simulink library "AFCToolbox"  (R2025b)
settings: Solver=VariableStepAuto  StartTime=0.0  StopTime=10.0  RelTol=1e-3
undefined symbols (not defined in the file or in its folder): AFC5Toolbox_SimuMoudle, ax, ay, az, C_d, C_dm, C_m, C_t, Control, d, declination_table, dp0, dp1, dp2, dp3, dt, euler_0, g0, I_xyz, inclination_table, J_m, lmd_high, lmd_low, lp_acc_knoise, lp_acc_max, lp_acc_min, lp_acc_seed, lp_GPS_BL_max, lp_GPS_BL_min, lp_GPS_H_max, lp_GPS_H_min, lp_GPS_knoise, lp_GPS_seed, lp_GPS_vel_max, lp_GPS_vel_min, lp_gyro_knoise, lp_gyro_max, lp_gyro_min, lp_gyro_seed, lp_hf_vwind, lp_hs_vwind_interp, lp_kaerorho, lp_kaeroT, lp_kIxyz, lp_kmass, lp_momentx_A0, lp_momentx_Af, lp_momentx_ts, lp_momenty_A0, lp_momenty_Af, lp_momenty_ts, lp_momentz_A0, lp_momentz_Af, lp_momentz_ts, lp_vf_vwind, lp_vs_vwind_interp, lp_vwind_thetax, lp_vwind_thetaz, mass, MB_states ... (+52)
libraries: $bdroot x104, simulink x75, etargetslib x32, sharedtransform x13, simulink_extras x12, dspstat3 x11, aerolibconvert2 x9, aerolibtransform2 x3, aerolibutil x2, matrix_library x1
(part 8 of 11)

== system AFCToolbox/SimuMoudle/UAV/Forces & Moments/Parameters/Air Parameter1/Air Model/W zhishu ==
  note: 1
  note: 2
  note: 3
  note: 4
  note: 5
  note: 6
  note: 7
  note: 8
  Z : Inport
  1 : Switch  Threshold=11.0191  SaturateOnIntegerOverflow=off  InputSameDT=off
  2 : Switch  Threshold=20.0631  SaturateOnIntegerOverflow=off  InputSameDT=off
  3 : Switch  Threshold=32.1619  SaturateOnIntegerOverflow=off  InputSameDT=off
  4 : Switch  Threshold=47.3501  SaturateOnIntegerOverflow=off  InputSameDT=off
  5 : Switch  Threshold=51.4125  SaturateOnIntegerOverflow=off  InputSameDT=off
  6 : Switch  Threshold=71.8020  SaturateOnIntegerOverflow=off  InputSameDT=off
  7 : Switch  Threshold=86  SaturateOnIntegerOverflow=off  InputSameDT=off
  constant1 : Constant  Value=11.2011
  constant10 : Constant
  constant11 : Constant  Value=-13.2011
  constant4 : Constant  Value=16.0816
  constant6 : Constant
  constant7 : Constant  Value=4.2559
  constant8 : Constant
  constant9 : Constant  Value=-35.1629
  zhishu : Outport
  wires:
  constant7/1 -> 1/3
  constant8/1 -> 1/1
  constant9/1 -> 2/1
  1/1 -> 2/3
  constant11/1 -> 3/1
  2/1 -> 3/3
  constant10/1 -> 4/1
  3/1 -> 4/3
  constant1/1 -> 5/1
  4/1 -> 5/3
  constant4/1 -> 6/1
  5/1 -> 6/3
  constant6/1 -> 7/1
  6/1 -> 7/3
  Z/1 -> 2/2, 6/2, 7/2, 5/2, 1/2, 3/2, 4/2
  7/1 -> zhishu/1

== system AFCToolbox/SimuMoudle/UAV/Forces & Moments/Parameters/Air Parameter1/Air Model/W zhishu1 ==
  note: 8
  note: 7
  note: 6
  note: 5
  note: 4
  note: 3
  note: 2
  note: 1
  Z : Inport
  1 : Switch  Threshold=11.0191  SaturateOnIntegerOverflow=off  InputSameDT=off
  2 : Switch  Threshold=20.0631  SaturateOnIntegerOverflow=off  InputSameDT=off
  3 : Switch  Threshold=32.1619  SaturateOnIntegerOverflow=off  InputSameDT=off
  4 : Switch  Threshold=47.3501  SaturateOnIntegerOverflow=off  InputSameDT=off
  5 : Switch  Threshold=51.4125  SaturateOnIntegerOverflow=off  InputSameDT=off
  6 : Switch  Threshold=71.8020  SaturateOnIntegerOverflow=off  InputSameDT=off
  7 : Switch  Threshold=86  SaturateOnIntegerOverflow=off  InputSameDT=off
  constant1 : Constant  Value=12.2011
  constant10 : Constant
  constant11 : Constant  Value=-12.2011
  constant4 : Constant  Value=17.0816
  constant6 : Constant
  constant7 : Constant  Value=5.2559
  constant8 : Constant
  constant9 : Constant  Value=-34.1629
  zhishu : Outport
  wires:
  7/1 -> zhishu/1
  Z/1 -> 4/2, 3/2, 1/2, 5/2, 7/2, 6/2, 2/2
  6/1 -> 7/3
  constant6/1 -> 7/1
  5/1 -> 6/3
  constant4/1 -> 6/1
  4/1 -> 5/3
  constant1/1 -> 5/1
  3/1 -> 4/3
  constant10/1 -> 4/1
  2/1 -> 3/3
  constant11/1 -> 3/1
  1/1 -> 2/3
  constant9/1 -> 2/1
  constant8/1 -> 1/1
  constant7/1 -> 1/3

== system AFCToolbox/SimuMoudle/UAV/Forces & Moments/Parameters/Air Parameter1/Air Model/rho xishu ==
  note: 8
  note: 7
  note: 6
  note: 5
  note: 4
  note: 3
  note: 2
  note: 1
  note: 9
  Z : Inport
  1 : Switch  Threshold=11.0191  SaturateOnIntegerOverflow=off  InputSameDT=off
  2 : Switch  Threshold=20.0631  SaturateOnIntegerOverflow=off  InputSameDT=off
  3 : Switch  Threshold=32.1619  SaturateOnIntegerOverflow=off  InputSameDT=off
  4 : Switch  Threshold=47.3501  SaturateOnIntegerOverflow=off  InputSameDT=off
  5 : Switch  Threshold=51.4125  SaturateOnIntegerOverflow=off  InputSameDT=off
  6 : Switch  Threshold=71.8020  SaturateOnIntegerOverflow=off  InputSameDT=off
  7 : Switch  Threshold=86  SaturateOnIntegerOverflow=off  InputSameDT=off
  8 : Switch  Threshold=91  SaturateOnIntegerOverflow=off  InputSameDT=off
  constant1 : Constant  Value=2.5280e-4
  constant10 : Constant  Value=9.4920e-4
  constant11 : Constant  Value=3.2618e-3
  constant2 : Constant  Value=0
  constant4 : Constant  Value=1.7632e-5
  constant6 : Constant  Value=3.6411e-6
  constant7 : Constant
  constant8 : Constant  Value=1.5898e-1
  constant9 : Constant  Value=3.2722e-2
  xishu : Outport
  wires:
  Z/1 -> 4/2, 3/2, 1/2, 5/2, 6/2, 7/2, 8/2, 2/2
  6/1 -> 7/3
  constant6/1 -> 7/1
  5/1 -> 6/3
  constant4/1 -> 6/1
  4/1 -> 5/3
  constant1/1 -> 5/1
  3/1 -> 4/3
  constant10/1 -> 4/1
  2/1 -> 3/3
  constant11/1 -> 3/1
  1/1 -> 2/3
  constant9/1 -> 2/1
  constant8/1 -> 1/1
  constant7/1 -> 1/3
  constant2/1 -> 8/1
  7/1 -> 8/3
  8/1 -> xishu/1

== system AFCToolbox/基础导航算法模型库/ECL EKF/init_state/State_mag1/Subsystem1/Subsystem/round down1 ==
  lat : Inport
  Data Type Conversion2 : DataTypeConversion  OutDataTypeStr=single  SaturateOnIntegerOverflow=off  RndMeth=Floor
  Floor2 : Rounding
  rad_to_index2 : Gain  Gain=0.1  OutDataTypeStr=int32
  rad_to_index3 : Gain  Gain=10  OutDataTypeStr=int32
  min_lat : Outport
  wires:
  Floor2/1 -> rad_to_index3/1
  lat/1 -> rad_to_index2/1
  rad_to_index3/1 -> min_lat/1
  rad_to_index2/1 -> Data Type Conversion2/1
  Data Type Conversion2/1 -> Floor2/1

== system AFCToolbox/基础导航算法模型库/ECL EKF/init_state/State_mag1/Subsystem1/Subsystem/round down3 ==
  lon : Inport
  Data Type Conversion2 : DataTypeConversion  OutDataTypeStr=single  SaturateOnIntegerOverflow=off  RndMeth=Floor
  Floor2 : Rounding
  rad_to_index2 : Gain  Gain=0.1  OutDataTypeStr=int32
  rad_to_index3 : Gain  Gain=10  OutDataTypeStr=int32
  min_lon : Outport
  wires:
  Floor2/1 -> rad_to_index3/1
  rad_to_index3/1 -> min_lon/1
  rad_to_index2/1 -> Data Type Conversion2/1
  lon/1 -> rad_to_index2/1
  Data Type Conversion2/1 -> Floor2/1

== system AFCToolbox/基础导航算法模型库/ECL EKF/init_state/State_mag1/Subsystem1/Subsystem2/round down1 ==
  lat : Inport
  Data Type Conversion2 : DataTypeConversion  OutDataTypeStr=single  SaturateOnIntegerOverflow=off  RndMeth=Floor
  Floor2 : Rounding
  rad_to_index2 : Gain  Gain=0.1  OutDataTypeStr=int32
  rad_to_index3 : Gain  Gain=10  OutDataTypeStr=int32
  min_lat : Outport
  wires:
  Data Type Conversion2/1 -> Floor2/1
  rad_to_index2/1 -> Data Type Conversion2/1
  rad_to_index3/1 -> min_lat/1
  lat/1 -> rad_to_index2/1
  Floor2/1 -> rad_to_index3/1

== system AFCToolbox/基础导航算法模型库/ECL EKF/init_state/State_mag1/Subsystem1/Subsystem2/round down3 ==
  lon : Inport
  Data Type Conversion2 : DataTypeConversion  OutDataTypeStr=single  SaturateOnIntegerOverflow=off  RndMeth=Floor
  Floor2 : Rounding
  rad_to_index2 : Gain  Gain=0.1  OutDataTypeStr=int32
  rad_to_index3 : Gain  Gain=10  OutDataTypeStr=int32
  min_lon : Outport
  wires:
  Data Type Conversion2/1 -> Floor2/1
  lon/1 -> rad_to_index2/1
  rad_to_index2/1 -> Data Type Conversion2/1
  rad_to_index3/1 -> min_lon/1
  Floor2/1 -> rad_to_index3/1

== system AFCToolbox/基础导航算法模型库/ECL EKF/init_state/State_mag1/Subsystem1/Subsystem3/round down1 ==
  lat : Inport
  Data Type Conversion2 : DataTypeConversion  OutDataTypeStr=single  SaturateOnIntegerOverflow=off  RndMeth=Floor
  Floor2 : Rounding
  rad_to_index2 : Gain  Gain=0.1  OutDataTypeStr=int32
  rad_to_index3 : Gain  Gain=10  OutDataTypeStr=int32
  min_lat : Outport
  wires:
  Data Type Conversion2/1 -> Floor2/1
  rad_to_index2/1 -> Data Type Conversion2/1
  rad_to_index3/1 -> min_lat/1
  lat/1 -> rad_to_index2/1
  Floor2/1 -> rad_to_index3/1

== system AFCToolbox/基础导航算法模型库/ECL EKF/init_state/State_mag1/Subsystem1/Subsystem3/round down3 ==
  lon : Inport
  Data Type Conversion2 : DataTypeConversion  OutDataTypeStr=single  SaturateOnIntegerOverflow=off  RndMeth=Floor
  Floor2 : Rounding
  rad_to_index2 : Gain  Gain=0.1  OutDataTypeStr=int32
  rad_to_index3 : Gain  Gain=10  OutDataTypeStr=int32
  min_lon : Outport
  wires:
  Data Type Conversion2/1 -> Floor2/1
  lon/1 -> rad_to_index2/1
  rad_to_index2/1 -> Data Type Conversion2/1
  rad_to_index3/1 -> min_lon/1
  Floor2/1 -> rad_to_index3/1

== matlab function AFCToolbox/ServoCardModule/XSrvoSamp/MATLAB Function ==
  data: ID1 input; out1 output; angleACK1 input; ID2 input; angleACK2 input; ID3 input; angleACK3 input; ID4 input; angleACK4 input; out2 output; out3 output; out4 output
function [out1, out2, out3, out4] = routeByID(ID1, angleACK1, ID2, angleACK2, ID3, angleACK3, ID4, angleACK4)
    % 1. 初始化输出数组（4个元素，对应Mux1-4号端口，默认0）
    out_array = zeros(1, 4);  % [out1, out2, out3, out4]
    
    % 2. 打包所有ID和angleACK为数组（批量处理，避免重复代码）
    IDs = [ID1, ID2, ID3, ID4];          % 所有ID的数组
    angles = [angleACK1, angleACK2, angleACK3, angleACK4];  % 所有角度的数组
    
    % 3. 循环遍历：ID在1-4范围内才赋值（索引直接对应端口）
    for i = 1:4
        id = IDs(i);
        if id >= 1 && id <= 4  % 仅处理合法ID（1-4）
            out_array(id) = angles(i);  % 关键：ID=1→out_array(1)=out1，直接索引赋值！
        end
    end
    
    % 4. 拆分输出数组为4个端口（对应Mux1-4号）
    [out1, out2, out3, out4] = deal(out_array(1), out_array(2), out_array(3), out_array(4));
end

== matlab function AFCToolbox/SimuMoudle/Position-Control/Consistent formation control /一致性控制——F2/MATLAB Function1 ==
  data: r input; result output
function result = Faixy(r)
%UNTITLED 此处显示有关此函数的摘要


result=-1.8*(1-exp(-0.5*r))/(1+exp(-0.5*r));



end

== matlab function AFCToolbox/SimuMoudle/Position-Control/Consistent formation control /一致性控制——F3/MATLAB Function2 ==
  data: r input; result output
function result = Faixy(r)
%UNTITLED 此处显示有关此函数的摘要


result=-1.8*(1-exp(-0.5*r))/(1+exp(-0.5*r));



end

== matlab function AFCToolbox/SimuMoudle/Position-Control/Consistent formation control /一致性控制——F1/Subsystem1/MATLAB Function ==
  data: i input; wx output; dt input; wy output
function [wx,wy] = w_error(i,dt)
%W_ERROR 此处显示有关此函数的摘要
%   此处显示详细说明
wx = 0.1*(cos(i*dt+pi/6)+cos(i*dt/3+pi/6)+cos(i*dt/5+pi/6)+cos(i*dt/7+pi/6));
wy = 0.1*(sin(i*dt+pi/6)+sin(i*dt/3+pi/6)+sin(i*dt/5+pi/6)+sin(i*dt/7+pi/6));

end

== matlab function AFCToolbox/SimuMoudle/Position-Control/Consistent formation control /一致性控制——F2/Subsystem2/MATLAB Function ==
  data: i input; wx output; dt input; wy output
function [wx,wy] = w_error(i,dt)
%W_ERROR 此处显示有关此函数的摘要
%   此处显示详细说明
wx = 0.1*(cos(i*dt+pi/6)+cos(i*dt/3+pi/6)+cos(i*dt/5+pi/6)+cos(i*dt/7+pi/6));
wy = 0.1*(sin(i*dt+pi/6)+sin(i*dt/3+pi/6)+sin(i*dt/5+pi/6)+sin(i*dt/7+pi/6));

end

== matlab function AFCToolbox/SimuMoudle/Position-Control/Consistent formation control /一致性控制——F3/Subsystem1/MATLAB Function ==
  data: i input; wx output; dt input; wy output
function [wx,wy] = w_error(i,dt)
%W_ERROR 此处显示有关此函数的摘要
%   此处显示详细说明
wx = 0.1*(cos(i*dt+pi/6)+cos(i*dt/3+pi/6)+cos(i*dt/5+pi/6)+cos(i*dt/7+pi/6));
wy = 0.1*(sin(i*dt+pi/6)+sin(i*dt/3+pi/6)+sin(i*dt/5+pi/6)+sin(i*dt/7+pi/6));

end

== matlab function AFCToolbox/SimuMoudle/Position-Control/Consistent formation control /一致性控制——F2/MATLAB Function2 ==
  data: r input; result output
function result = Faixy(r)
%UNTITLED 此处显示有关此函数的摘要


result=-1.8*(1-exp(-0.5*r))/(1+exp(-0.5*r));



end

== matlab function AFCToolbox/SimuMoudle/Position-Control/Consistent formation control /一致性控制——F1/MATLAB Function1 ==
  data: r input; result output
function result = Faixy(r)
%UNTITLED 此处显示有关此函数的摘要


result=-1.8*(1-exp(-0.5*r))/(1+exp(-0.5*r));



end

== matlab function AFCToolbox/SimuMoudle/Position-Control/Consistent formation control /一致性控制——F1/MATLAB Function2 ==
  data: r input; result output
function result = Faixy(r)
%UNTITLED 此处显示有关此函数的摘要


result=-1.8*(1-exp(-0.5*r))/(1+exp(-0.5*r));



end

== matlab function AFCToolbox/SimuMoudle/Position-Control/Consistent formation control /一致性控制——F1/MATLAB Function4 ==
  data: r input; result output
function result = Faixy(r)
%UNTITLED 此处显示有关此函数的摘要


result=-1.8*(1-exp(-0.5*r))/(1+exp(-0.5*r));



end

== matlab function AFCToolbox/SimuMoudle/Position-Control/Consistent formation control /一致性控制——F3/MATLAB Function3 ==
  data: r input; result output
function result = Faixy(r)
%UNTITLED 此处显示有关此函数的摘要


result=-1.8*(1-exp(-0.5*r))/(1+exp(-0.5*r));



end

== matlab function AFCToolbox/SimuMoudle/Position-Control/Leader/Subsystem/Follower1/MATLAB Function ==
  data: theta input; J output; phi input; v input
function J = TA_xyz(theta,phi,v)
a=cos(theta)*cos(phi);
b=-v*sin(theta)*cos(phi);
c=-v*cos(theta)*sin(phi);

d=sin(theta)*cos(phi);
e=v*cos(theta)*cos(phi);
f=-v*sin(theta)*sin(phi);

g=sin(phi);
h=0;
i=v*cos(phi);

J=[a,b,c;
    d,e,f;
    g,h,i];
end

== matlab function AFCToolbox/SimuMoudle/Position-Control/Leader/Subsystem/Follower1/MATLAB Function1 ==
  data: W input; result output
function result = Faiv(W)
%UNTITLED 此处显示有关此函数的摘要


result=-0.5*(1-exp(-0.5*W))/(1+exp(-0.5*W));



end

== matlab function AFCToolbox/SimuMoudle/Position-Control/Leader/Subsystem/Follower1/MATLAB Function2 ==
  data: w input; result output
function result = Faiv(w)
%UNTITLED 此处显示有关此函数的摘要


result=-0.5*(1-exp(-0.5*w))/(1+exp(-0.5*w));



end

== matlab function AFCToolbox/SimuMoudle/Position-Control/Leader/Subsystem/Follower1/MATLAB Function3 ==
  data: r input; result output
function result = Faiv(r)
%UNTITLED 此处显示有关此函数的摘要


result=-0.5*(1-exp(-0.5*r))/(1+exp(-0.5*r));



end

== matlab function AFCToolbox/SimuMoudle/Position-Control/Leader/Subsystem/Follower2/MATLAB Function ==
  data: theta input; J output; phi input; v input
function J = TA_xyz(theta,phi,v)
a=cos(theta)*cos(phi);
b=-v*sin(theta)*cos(phi);
c=-v*cos(theta)*sin(phi);

d=sin(theta)*cos(phi);
e=v*cos(theta)*cos(phi);
f=-v*sin(theta)*sin(phi);

g=sin(phi);
h=0;
i=v*cos(phi);

J=[a,b,c;
    d,e,f;
    g,h,i];
end

== matlab function AFCToolbox/SimuMoudle/Position-Control/Leader/Subsystem/Follower2/MATLAB Function1 ==
  data: W input; result output
function result = Faiv(W)
%UNTITLED 此处显示有关此函数的摘要


result=-0.5*(1-exp(-0.5*W))/(1+exp(-0.5*W));



end

== matlab function AFCToolbox/SimuMoudle/Position-Control/Leader/Subsystem/Follower2/MATLAB Function2 ==
  data: w input; result output
function result = Faiv(w)
%UNTITLED 此处显示有关此函数的摘要


result=-0.5*(1-exp(-0.5*w))/(1+exp(-0.5*w));



end

== matlab function AFCToolbox/SimuMoudle/Position-Control/Leader/Subsystem/Follower2/MATLAB Function3 ==
  data: r input; result output
function result = Faiv(r)
%UNTITLED 此处显示有关此函数的摘要


result=-0.5*(1-exp(-0.5*r))/(1+exp(-0.5*r));



end

== matlab function AFCToolbox/SimuMoudle/Position-Control/Leader/Subsystem/Follower3/MATLAB Function ==
  data: theta input; J output; phi input; v input
function J = TA_xyz(theta,phi,v)
a=cos(theta)*cos(phi);
b=-v*sin(theta)*cos(phi);
c=-v*cos(theta)*sin(phi);

d=sin(theta)*cos(phi);
e=v*cos(theta)*cos(phi);
f=-v*sin(theta)*sin(phi);

g=sin(phi);
h=0;
i=v*cos(phi);

J=[a,b,c;
    d,e,f;
    g,h,i];
end

== matlab function AFCToolbox/SimuMoudle/Position-Control/Leader/Subsystem/Follower3/MATLAB Function1 ==
  data: W input; result output
function result = Faiv(W)
%UNTITLED 此处显示有关此函数的摘要


result=-0.5*(1-exp(-0.5*W))/(1+exp(-0.5*W));



end

== stateflow chart AFCToolbox/SimuMoudle/UAV/Equations of Motion/Chart ==
  state Land
    en, du: ground_contact = 1;
  state Flight
    en, du: ground_contact = 0;
  (default) -> Land
  Flight -> Land : [h<=0 && vel(3) >0]
  Land -> Flight : [acc(3)<0]
  data: h input; vel input; acc input; ground_contact output

== matlab function AFCToolbox/SimuMoudle/Position-Control/Leader/Subsystem/Follower3/MATLAB Function2 ==
  data: w input; result output
function result = Faiv(w)
%UNTITLED 此处显示有关此函数的摘要


result=-0.5*(1-exp(-0.5*w))/(1+exp(-0.5*w));



end

== matlab function AFCToolbox/SimuMoudle/Position-Control/Leader/Subsystem/Follower3/MATLAB Function3 ==
  data: r input; result output
function result = Faiv(r)
%UNTITLED 此处显示有关此函数的摘要


result=-0.5*(1-exp(-0.5*r))/(1+exp(-0.5*r));



end

== matlab function AFCToolbox/SimuMoudle/SimuGps/LLA model/Subsystem1/ECEF地心坐标系-经纬高 ==
  data: x input; l output; y input; z input; b output; h output
function [l,b,h] = fcn(x,y,z)
[l,b,h] = xyz2lbh(x,y,z);

== matlab function AFCToolbox/SimuMoudle/Position-Control/Consistent formation control /一致性控制——F3/MATLAB Function1 ==
  data: r input; result output
function result = Faixy(r)
%UNTITLED 此处显示有关此函数的摘要


result=-1.8*(1-exp(-0.5*r))/(1+exp(-0.5*r));



end

== matlab function AFCToolbox/SimuMoudle/SimuGps/LLA model/Subsystem1/北天东-ECEF地心坐标系 ==
  data: pn input; DX output; ph input; pe input; Lon0 input; Lat0 input; Alt0 input; DY output; DZ output
function [ DX,DY,DZ ] = TransformBTD_T_DX( pn,ph,pe,Lon0,Lat0,Alt0 )
%TransformBTDTDX 此处显示有关此函数的摘要
%将北天东系转换到地心坐标系
m_dN_LE = zeros(3,3);

[ DX0,DY0,DZ0 ] = TransformLLA_T_DX(Lon0,Lat0,Alt0);%经纬高转为地面坐标系G

Fai = Lat0;
Lamda = Lon0;

x_bt = pn;
y_bt = ph;
z_bt = pe;

m_dN_LE(1,1) = -sin(Fai)*cos(Lamda);
m_dN_LE(1,2) = cos(Fai)*cos(Lamda);
m_dN_LE(1,3) = -sin(Lamda);
m_dN_LE(2,1) = -sin(Fai)*sin(Lamda);
m_dN_LE(2,2) = cos(Fai)*sin(Lamda);
m_dN_LE(2,3) = cos(Lamda);
m_dN_LE(3,1) = cos(Fai);
m_dN_LE(3,2) = sin(Fai);
m_dN_LE(3,3) = 0.0;

A = m_dN_LE*[x_bt;y_bt;z_bt];
x_dx = A(1);
y_dx = A(2);
z_dx = A(3);

DX = DX0 + x_dx;
DY = DY0 + y_dx;
DZ = DZ0 + z_dx;

end

== matlab function AFCToolbox/SimuMoudle/SimuICM/acclerate  model2/Subsystem/MATLAB Function ==
  data: accBias input; accData output; correlationTimeConstant input; accNoiseStdDev input; dt input
function accData= fcn(accBias,correlationTimeConstant,accNoiseStdDev,dt)
persistent initaccBias;

%单位换算
arcdeg = pi/180;hur = 3600;dph = arcdeg / hur;Hz = 1;g=9.7803267714;
% accNoiseStdDev = 100;           % 加速度一阶马尔可夫噪声均方根ug
% accBiasOffsetStdDev =100;      % 陀螺仪零偏漂移标准差ug
% 
% %常值漂移
% eb = accBiasOffsetStdDev * g * randn(1,1);

%一阶马尔可夫相关时间T;反相关时间beta = 1/T;
% TauG = 3600;
beta = 1/correlationTimeConstant; 
% 方差R0（m/s^2）
R0 = (accNoiseStdDev*g)^2;

%角速率随机游走系数
q = 2*beta*R0;


if isempty(initaccBias)
    initaccBias = sqrt(R0)*randn(1,1);
    accBias= initaccBias;
end

 
Phi = 1 -beta*dt;
sQkr =sqrt(q*dt);
accBias=Phi*accBias+sQkr*randn(1,1);
% 生成加速度数据
accData =  accBias;
end

== matlab function AFCToolbox/SimuMoudle/SimuICM/acclerate  model2/Subsystem1/MATLAB Function ==
  data: accBias input; accData output; correlationTimeConstant input; accNoiseStdDev input; dt input
function accData= fcn(accBias,correlationTimeConstant,accNoiseStdDev,dt)
persistent initaccBias;

%单位换算
arcdeg = pi/180;hur = 3600;dph = arcdeg / hur;Hz = 1;g=9.7803267714;
% accNoiseStdDev = 100;           % 加速度一阶马尔可夫噪声均方根ug
% accBiasOffsetStdDev =100;      % 陀螺仪零偏漂移标准差ug
% 
% %常值漂移
% eb = accBiasOffsetStdDev * g * randn(1,1);

%一阶马尔可夫相关时间T;反相关时间beta = 1/T;
% TauG = 3600;
beta = 1/correlationTimeConstant; 
% 方差R0（m/s^2）
R0 = (accNoiseStdDev*g)^2;

%角速率随机游走系数
q = 2*beta*R0;


if isempty(initaccBias)
    initaccBias = sqrt(R0)*randn(1,1);
    accBias= initaccBias;
end

 
Phi = 1 -beta*dt;
sQkr =sqrt(q*dt);
accBias=Phi*accBias+sQkr*randn(1,1);
% 生成加速度数据
accData =  accBias;
end

== matlab function AFCToolbox/SimuMoudle/SimuICM/acclerate  model2/Subsystem2/MATLAB Function ==
  data: accBias input; accData output; correlationTimeConstant input; accNoiseStdDev input; dt input
function accData= fcn(accBias,correlationTimeConstant,accNoiseStdDev,dt)
persistent initaccBias;

%单位换算
arcdeg = pi/180;hur = 3600;dph = arcdeg / hur;Hz = 1;g=9.7803267714;
% accNoiseStdDev = 100;           % 加速度一阶马尔可夫噪声均方根ug
% accBiasOffsetStdDev =100;      % 陀螺仪零偏漂移标准差ug
% 
% %常值漂移
% eb = accBiasOffsetStdDev * g * randn(1,1);

%一阶马尔可夫相关时间T;反相关时间beta = 1/T;
% TauG = 3600;
beta = 1/correlationTimeConstant; 
% 方差R0（m/s^2）
R0 = (accNoiseStdDev*g)^2;

%角速率随机游走系数
q = 2*beta*R0;


if isempty(initaccBias)
    initaccBias = sqrt(R0)*randn(1,1);
    accBias= initaccBias;
end

 
Phi = 1 -beta*dt;
sQkr =sqrt(q*dt);
accBias=Phi*accBias+sQkr*randn(1,1);
% 生成加速度数据
accData =  accBias;
end

== matlab function AFCToolbox/SimuMoudle/SimuICM/gyro model1/Subsystem/MATLAB Function ==
  data: gyroBias input; gyroData output; correlationTimeConstant input; gyroNoiseStdDev input; dt input
function gyroData= fcn(gyroBias,correlationTimeConstant,gyroNoiseStdDev,dt)
persistent initgyroBias;

%单位换算
arcdeg = pi/180;hur = 3600;dph = arcdeg / hur;Hz = 1;
% gyroNoiseStdDev = 0.1;           % 陀螺仪一阶马尔可夫噪声均方根°/h
% gyroBiasOffsetStdDev = 0.1;      % 陀螺仪零偏漂移标准差rad/s
% 
% %常值漂移
% eb = gyroBiasOffsetStdDev * dph * randn(1,1);

%一阶马尔可夫相关时间T;反相关时间beta = 1/T;
% TauG = 3600;
beta = 1/correlationTimeConstant; 
% 方差R0（rad/s）
R0 = (gyroNoiseStdDev*dph)^2;

%角速率随机游走系数
q = 2*beta*R0;


if isempty(initgyroBias)
    initgyroBias = sqrt(R0)*randn(1,1);
    gyroBias= initgyroBias;
end

 
Phi = 1 -beta*dt;
sQkr =sqrt(q*dt);
gyroBias=Phi*gyroBias+sQkr*randn(1,1);
% 生成陀螺仪数据
gyroData =  gyroBias;
end

== matlab function AFCToolbox/SimuMoudle/SimuICM/gyro model1/Subsystem1/MATLAB Function ==
  data: gyroBias input; gyroData output; correlationTimeConstant input; gyroNoiseStdDev input; dt input
function gyroData= fcn(gyroBias,correlationTimeConstant,gyroNoiseStdDev,dt)
persistent initgyroBias;

%单位换算
arcdeg = pi/180;hur = 3600;dph = arcdeg / hur;Hz = 1;
% gyroNoiseStdDev = 0.1;           % 陀螺仪一阶马尔可夫噪声均方根°/h
% gyroBiasOffsetStdDev = 0.1;      % 陀螺仪零偏漂移标准差rad/s
% 
% %常值漂移
% eb = gyroBiasOffsetStdDev * dph * randn(1,1);

%一阶马尔可夫相关时间T;反相关时间beta = 1/T;
% TauG = 3600;
beta = 1/correlationTimeConstant; 
% 方差R0（rad/s）
R0 = (gyroNoiseStdDev*dph)^2;

%角速率随机游走系数
q = 2*beta*R0;


if isempty(initgyroBias)
    initgyroBias = sqrt(R0)*randn(1,1);
    gyroBias= initgyroBias;
end

 
Phi = 1 -beta*dt;
sQkr =sqrt(q*dt);
gyroBias=Phi*gyroBias+sQkr*randn(1,1);
% 生成陀螺仪数据
gyroData =  gyroBias;
end

== matlab function AFCToolbox/SimuMoudle/Position-Control/Leader/MATLAB Function ==
  data: theta input; J output; phi input; v input
function J = TA_xyz(theta,phi,v)
a=cos(theta)*cos(phi);
b=-v*sin(theta)*cos(phi);
c=-v*cos(theta)*sin(phi);

d=sin(theta)*cos(phi);
e=v*cos(theta)*cos(phi);
f=-v*sin(theta)*sin(phi);

g=sin(phi);
h=0;
i=v*cos(phi);

J=[a,b,c;
    d,e,f;
    g,h,i];
end

== matlab function AFCToolbox/SimuMoudle/SimuICM/gyro model1/Subsystem2/MATLAB Function ==
  data: gyroBias input; gyroData output; correlationTimeConstant input; gyroNoiseStdDev input; dt input
function gyroData= fcn(gyroBias,correlationTimeConstant,gyroNoiseStdDev,dt)
persistent initgyroBias;

%单位换算
arcdeg = pi/180;hur = 3600;dph = arcdeg / hur;Hz = 1;
% gyroNoiseStdDev = 0.1;           % 陀螺仪一阶马尔可夫噪声均方根°/h
% gyroBiasOffsetStdDev = 0.1;      % 陀螺仪零偏漂移标准差rad/s
% 
% %常值漂移
% eb = gyroBiasOffsetStdDev * dph * randn(1,1);

%一阶马尔可夫相关时间T;反相关时间beta = 1/T;
% TauG = 3600;
beta = 1/correlationTimeConstant; 
% 方差R0（rad/s）
R0 = (gyroNoiseStdDev*dph)^2;

%角速率随机游走系数
q = 2*beta*R0;


if isempty(initgyroBias)
    initgyroBias = sqrt(R0)*randn(1,1);
    gyroBias= initgyroBias;
end

 
Phi = 1 -beta*dt;
sQkr =sqrt(q*dt);
gyroBias=Phi*gyroBias+sQkr*randn(1,1);
% 生成陀螺仪数据
gyroData =  gyroBias;
end

== matlab function AFCToolbox/SimuMoudle/SimuBaro/Baro model/MATLAB Function ==
  data: h input; P output
function P = altitude_to_pressure(h)
    % 输入：高度 h（单位：米）
    % 输出：压强 P（单位：Pa）

    % 常量定义
    P0 = 101325;  % 海平面上的大气压强，单位Pa
    L = 0.0065;   % 温度递减率，单位K/m
    T0 = 288.15;  % 海平面上的温度，单位K
    g0 = 9.80665; % 重力加速度，单位m/s²
    M = 0.0289644; % 空气摩尔质量，单位kg/mol
    R = 8.314462618; % 气体常数，单位J/(mol·K)

    % 计算压强
    P = P0 * (1 - (L * h) / T0)^(g0 * M / (R * L));
end

== matlab function AFCToolbox/SimuMoudle/SimuBaro/Baro model/MATLAB Function1 ==
  data: altitude input; pressure output; temperature output
function [pressure, temperature] = calculateAtmosphereProperties(altitude)
    % 标准大气参数
    R = 287; % 干空气的特定气体常数，单位 J/(kg*K)
    g = 9.81; % 重力加速度，单位 m/s^2
    T0 = 293.15; % 海平面标准温度，单位 K
    p0 = 101325; % 海平面标准压强，单位 Pa
    lapserate = -0.0065; % 环境递减率，单位 K/m

    % 计算给定高度的压强和温度
    if altitude <= 11000
        temperature = T0 + lapserate * altitude; % 温度随高度线性递减
    else
        temperature = T0 + lapserate * 11000; % 高于11公里后温度保持不变
    end
    pressure = p0 * (T0/temperature)^(-g/R/lapserate); % 压强随高度和温度变化

    % 输出结果
    pressure = pressure; % 返回压强
    
    % 将温度从开尔文转换为摄氏度
    temperature = temperature - 273.15;% 返回温度
end

== matlab function AFCToolbox/基础导航算法模型库/ECL EKF/Subsystem/InitCovariance1 ==
  data: covariance output; dt input
function covariance = InitCovariance(dt)
%% Initial Uncertainty
param.alignment.posErrNE = 10.0; % Initial 1SD position error when aligning without GPS. (m/sec)
param.alignment.velErrNE = 5.0; % Initial 1SD velocity error when aligning without GPS. (m/sec)
param.alignment.velErrD = 1.0; % Initial 1SD vertical velocity error when aligning without GPS. (m/sec)
param.alignment.delAngBiasErr = 0.05*pi/180; % Initial 1SD rate gyro bias uncertainty. (rad/sec)
param.alignment.delVelBiasErr = 0.07; % Initial 1SD accelerometer bias uncertainty. (m/sec^2)
param.alignment.quatErr = 0.01; % Initial 1SD uncertainty in quaternion.
param.alignment.magErrXYZ = 0.01; % Initial 1SD uncertainty in body frame XYZ magnetic field states. (gauss)
param.alignment.magErrNED = 0.5; % Initial 1SD uncertainty in earth frame NED magnetic field states. (gauss)
param.alignment.hgtErr = 0.5; % Initial 1SD uncertainty in height. (m)
param.alignment.windErrNE = 5.0; % Initial 1SD error in wind states. (m/sec)


% Define quaternion state errors
Sigma_quat = param.alignment.quatErr * [1;1;1;1];
% Define velocity state errors
Sigma_velocity = param.alignment.velErrNE * [1;1;1];

% Define position state errors
Sigma_position = param.alignment.posErrNE * [1;1;1];


% Define delta angle bias state errors
Sigma_dAngBias = param.alignment.delAngBiasErr*dt*[1;1;1];

% Define delta velocity bias state errors
Sigma_dVelBias = param.alignment.delVelBiasErr*dt*[1;1;1];

% Define magnetic field state errors
Sigma_magNED = [param.alignment.magErrNED;param.alignment.magErrNED;param.alignment.magErrNED]; % 1 Sigma uncertainty in initial NED mag field
Sigma_magXYZ = [param.alignment.magErrXYZ;param.alignment.magErrXYZ;param.alignment.magErrXYZ]; % 1 Sigma uncertainty in initial XYZ mag sensor offset

% Define wind velocity state errors
Sigma_wind = param.alignment.windErrNE * [1;1];

% Convert to variances and write to covariance matrix diagonals
covariance = diag([Sigma_quat;Sigma_velocity;Sigma_position;Sigma_dAngBias;Sigma_dVelBias;Sigma_magNED;Sigma_magXYZ;Sigma_wind].^2);
end

== matlab function AFCToolbox/基础导航算法模型库/ECL EKF/Subsystem/Mag Fusion/Control MagDeclination Fusion1 ==
  data: states input; states output; P input; R_decl input; measDec input; P output
function [...
    states, ... % state vector after fusion of measurements
    P] ... %
    = FuseMagDeclination( ...
    states, ... % state vector after fusion of measurements
    P, ... %
    R_decl,...
    measDec) % magnetic field declination - azimuth angle measured from true north (rad)

% magNE
magN = states(17);
magE = states(18);

H = zeros(1,24);
Kfusion = zeros(24,1);

R_DECL = R_decl^2;
	HK0 = power(magN, -2);
	HK1 = HK0*power(magE, 2) + 1.0;
	HK2 = 1.0/HK1;
	HK3 = 1.0/magN;
	HK4 = HK2*HK3;
    HK5 = HK3*magE;
	HK6 = HK5*P(17,18) - P(18,18);
	HK7 = power(HK1, -2);
	HK8 = HK5*P(17,17) - P(17,18);
    innovation_variance = -HK0*HK6*HK7 + HK7*HK8*magE/power(magN, 3) + R_DECL;
    HK9 = HK4/innovation_variance;

H(17) = -HK0*HK2*magE;
H(18) = HK4;

	for row = 1:16
		Kfusion(row) = -HK9*(HK5*P(row,17) - P(row,18));
    end

	Kfusion(17) = -HK8*HK9;
	Kfusion(18) = -HK6*HK9;

	for  row = 19:24
		Kfusion(row) = -HK9*(HK5*P(17,row) - P(18,row));
    end


% Magnetic declination noise R = σdelc^2
%R_MAG = 0.5^2;

%% Hψ_dec = ∂ψ_dec / ∂x
%H = calcH_MAGD(magE,magN);
% S = Hψ_dec * P * PT + R_MAG
%varInnov = (H*P*transpose(H) + R_MAG);
% Optimal Kalman gain, K = Pk+1|k * Hψ_dec / S
%Kfusion = (P*transpose(H))/varInnov;

% Calculate the predicted magnetic declination, ψ_dec = arctan(mE/mN)
predDec = atan2(magE,magN);

% Calculate the measurement innovation, yk = zψ_dec - ψ_dec
innovation = measDec- predDec;

if (innovation > 0.5)
    innovation = single(0.5);
elseif (innovation < -0.5)
    innovation = single(-0.5);
end

% correct the state vector, xk+1|k+1 = xk+1|k + K*yk
states = states + Kfusion * innovation;

% correct the covariance Pk+1|k+1 = Pk+1|k - K * Hψ_dec * Pk+1|k
%P = P - Kfusion*H*P;
KHP = computeKHP(Kfusion, H, P);
P = P - KHP;
%% Force symmetry on the covariance matrix to prevent ill-conditioning
% of the matrix which would cause the filter to blow-up
P = 0.5*(P + transpose(P));

% ensure diagonals are positive
for i=1:24
    if P(i,i) < 0
        P(i,i) = single(0);
    end
end
% fixCovarianceErrors(true);
% limitDeclination();
end
